simulink model "optimization_example"  (R2025b)
settings: Solver=VariableStepAuto  StartTime=0.0  StopTime=10  RelTol=1e-3
values from neighbouring files (symbols this model uses):
  N_units = 10    [opt_script.m]
libraries: customization_lib x8, fl_lib x1, nesl_utility x1
settings Model: Creator=degoede  LastModifiedBy=degoede
settings SimscapeCC: SimscapeLogSimulationStatistics=on  SimscapeLogOpenViewer=on

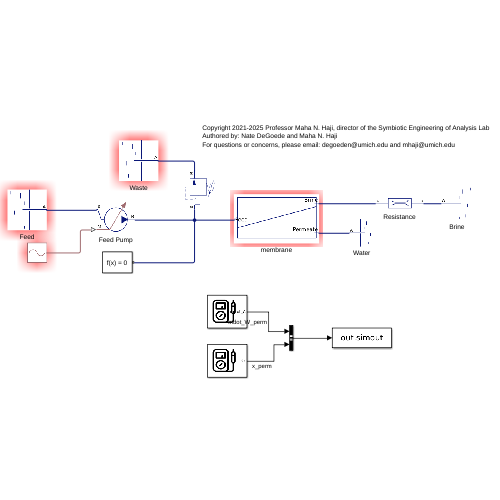
[thumbnail: Simulink's stored preview of the top-level diagram]
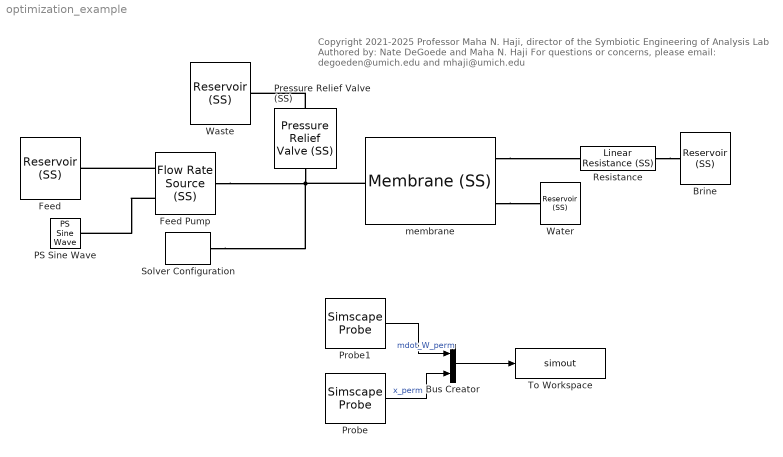
== system optimization_example ==
  note: Copyright 2021-2025 Professor Maha N. Haji, director of the Symbiotic Engineering of Analysis Lab
      | Authored by: Nate DeGoede and Maha N. Haji
      | For questions or concerns, please email: degoeden@umich.edu and mhaji@umich.edu
  Brine : customization_lib/solution/elements/Reservoir (SS)  pressure_spec=foundation.enum.pressure_spec.atmospheric  reservoir_pressure=0.101325 MPa  reservoir_temperature=293.15 K  reservoir_concentration=50 kg/m^3  area=27 mm^2
      settings: SourceProductName=Customization  InternalSimscapePortConfiguration="{\"Bottom\":[],\"Left\":[{\"id\":\"A\",\"label\":\"A\",\"type\":\"customization.solution.solution\"}],\"Right\":[],\"Top\":[]}"
  Bus Creator : BusCreator  Inputs=2
  Feed : customization_lib/solution/elements/Reservoir (SS)  pressure_spec=foundation.enum.pressure_spec.atmospheric  reservoir_pressure=P_feed MPa  reservoir_temperature=293.15 K  reservoir_concentration=x_feed kg/m^3  area=1 cm^2
      settings: SourceProductName=Customization  InternalSimscapePortConfiguration="{\"Bottom\":[],\"Left\":[{\"id\":\"A\",\"label\":\"A\",\"type\":\"customization.solution.solution\"}],\"Right\":[],\"Top\":[]}"
  Feed Pump : customization_lib/solution/sources/Flow Rate Source (SS)  source_type=foundation.enum.constant_controlled.controlled  flow_type=foundation.enum.mass_volumetric_flow.mass  mass_flow=0 kg/s  volumetric_flow=0 m^3/s  power_spec=foundation.enum.power_spec.isentropic  area=0.01 m^2
      settings: SourceProductName=Customization  InternalSimscapePortConfiguration="{\"Bottom\":[],\"Left\":[{\"id\":\"A\",\"label\":\"A\",\"type\":\"customization.solution.solution\"},{\"id\":\"M\",\"label\":\"M\",\"type\":\"input\"}],\"Right\":[{\"id\":\"B\",\"label\":\"B\",\"type\":\"customization.solution.solution\"}],\"Top\":[]}"
  PS Sine Wave : fl_lib/Physical Signals/Sources/PS Sine Wave  amplitude=mdot_amp kg/s  bias=mdot_mean kg/s  frequency_spec=foundation.enum.frequencySpec.frequencySI  frequency_SI=1 Hz  frequency_angular=1 rad/s  phase=0 rad
      settings: InternalSimscapePortConfiguration="{\"Bottom\":[],\"Left\":[],\"Right\":[{\"id\":\"O\",\"label\":\"\",\"type\":\"output\"}],\"Top\":[]}"
  Pressure Relief Valve (SS) : customization_lib/solution/elements/Pressure Relief Valve (SS)  set_pressure=6 MPa  reg_range=0.1 MPa  max_area=0.005 m^2  min_area=1e-10 m^2  area=0.01 m^2  Cd=0.64  Re_c=150
      settings: SourceProductName=Customization  InternalSimscapePortConfiguration="{\"Bottom\":[],\"Left\":[{\"id\":\"A\",\"label\":\"A\",\"type\":\"customization.solution.solution\"}],\"Right\":[{\"id\":\"B\",\"label\":\"B\",\"type\":\"customization.solution.solution\"}],\"Top\":[]}"
  Probe : SimscapeProbe  BoundBlock=34  Variables="{\"P.x\":{\"Probing\":\"ON\"}}"
  Probe1 : SimscapeProbe  BoundBlock=29  Variables="{\"mdot_A\":{\"Probing\":\"ON\"}}"
  Resistance : customization_lib/solution/elements/Linear Resistance (SS)  R=6200000000 Pa*s/m^3  area=0.01 m^2
      settings: SourceProductName=Customization  InternalSimscapePortConfiguration="{\"Bottom\":[],\"Left\":[{\"id\":\"A\",\"label\":\"A\",\"type\":\"customization.solution.solution\"}],\"Right\":[{\"id\":\"B\",\"label\":\"B\",\"type\":\"customization.solution.solution\"}],\"Top\":[]}"
  Solver Configuration : nesl_utility/Solver Configuration  PhysicalDomain=network_engine_domain  SubClassName=solver  LeftPortType=input  RightPortType=generic  Tones=[]  Harmonics=[]  SimulateNoise=off  Profile=off  UseLocalSampling=off  EnableSwitchedLinearOptims=on  FrequencyDomain=off  UseCCode=off  RelTol=0.001  AbsTol=0.001  MinStep=1e-09  ToWorkspace=off  RevertToSquareIcSolve=off  NumHomotopyIterations=100  PhasorMode=off  PhasorModeNumHarmonics=1  ConsistencySolver=NEWTON_XTOL_AFTER_FTOL  IndexReductionMethod=DerivativeReplacement  DoDC=off  ResidualTolerance=1e-09  ConsistencyTolSource=GLOBAL  ConsistencyAbsTol=0.001  ConsistencyRelTol=0.001  ConsistencyTolFactor=0.001  UseLocalSolver=off  LocalSolverChoice=NE_BACKWARD_EULER_ADVANCER  ResolveIndetEquations=on  FunctionEvalNumThread=1  LocalSolverSampleTime=0.001  DoFixedCost=off  MaxNonlinIter=3  MaxModeIter=2  ComputeImpulses=off  ImpulseIterations=2  LinearAlgebra=auto  LinearAlgebraNumThread=0  EquationFormulation=NE_TIME_EF  DelaysMemoryBudget=1024  AutomaticFiltering=off  FilteringTimeConstant=0.001  PartitionStorageMethod=AS_NEEDED  PartitionMemoryBudget=1024  PartitionMethod=ROBUST  MultibodyUseLocalSolver=off  MultibodyLocalSolverChoice=ODE1  MultibodyLocalSolverSampleTime=0.001
  To Workspace : ToWorkspace  VariableName=simout  SaveFormat=Timeseries  SampleTime=-1
  Waste : customization_lib/solution/elements/Reservoir (SS)  pressure_spec=foundation.enum.pressure_spec.atmospheric  reservoir_pressure=P_feed MPa  reservoir_temperature=293.15 K  reservoir_concentration=x_feed kg/m^3  area=1 cm^2
      settings: SourceProductName=Customization  InternalSimscapePortConfiguration="{\"Bottom\":[],\"Left\":[{\"id\":\"A\",\"label\":\"A\",\"type\":\"customization.solution.solution\"}],\"Right\":[],\"Top\":[]}"
  Water : customization_lib/solution/elements/Reservoir (SS)  pressure_spec=foundation.enum.pressure_spec.atmospheric  reservoir_pressure=0.101325 MPa  reservoir_temperature=293.15 K  reservoir_concentration=0 kg/m^3  area=1 cm^2
      settings: SourceProductName=Customization  InternalSimscapePortConfiguration="{\"Bottom\":[],\"Left\":[{\"id\":\"A\",\"label\":\"A\",\"type\":\"customization.solution.solution\"}],\"Right\":[],\"Top\":[]}"
  membrane : customization_lib/membranes/Membrane (SS)  A_w=A_w m^3/(N*s)  B_s=B_s m/s  A_m=35 m^2  length=1 m  D_feed=D_feed mm  area_feed=area_feed mm^2  D_perm=D_perm mm  N=N_units  P0_feed=P_feed MPa  P0_perm=0.101 MPa  x0_feed=x_feed kg/m^3  x0_perm=0 kg/m^3
      settings: SourceProductName=Customization  InternalSimscapePortConfiguration="{\"Bottom\":[],\"Left\":[{\"id\":\"F\",\"label\":\"Feed\",\"type\":\"customization.solution.solution\"}],\"Right\":[{\"id\":\"B\",\"label\":\"Brine\",\"type\":\"customization.solution.solution\"},{\"id\":\"P\",\"label\":\"Permeate\",\"type\":\"customization.solution.solution\"}],\"Top\":[]}"
  wires:
  Probe/1 -> Bus Creator/2  "x_perm"
  Bus Creator/1 -> To Workspace/1
  Probe1/1 -> Bus Creator/1  "mdot_W_perm"
  connections:
  Solver Configuration/RConn1 -- membrane/LConn1 -- Pressure Relief Valve (SS)/LConn1 -- Feed Pump/RConn1
  membrane/RConn1 -- Resistance/LConn1
  membrane/RConn2 -- Water/LConn1
  Resistance/RConn1 -- Brine/LConn1
  Feed Pump/LConn1 -- Feed/LConn1
  Feed Pump/LConn2 -- PS Sine Wave/RConn1
  Pressure Relief Valve (SS)/RConn1 -- Waste/LConn1
